simulink subsystem "BatteryHV_Primitive_refsub"  (R2025a)
settings: Solver=VariableStepAuto  StartTime=0.0  StopTime=10.0  RelTol=1e-3
undefined symbols (not defined in the file or in its folder): batteryHV, Minus, Plus
libraries: fl_lib x14, nesl_utility x6
settings Model: Creator=isaacito  LastModifiedBy=isaacito
settings SolverCC: AlgebraicLoopSolver=TrustRegion
settings OptimizationCC: ReuseModelBlockBuffer=off
settings DebuggingCC: UnconnectedInputMsg=warning  UnconnectedOutputMsg=warning  UnconnectedLineMsg=warning
settings ModelReferenceCC: EnableRefExpFcnMdlSchedulingChecks=on
settings RTWCC: GPUComputeCapability=3.5  DLArmComputeVersion=19.05

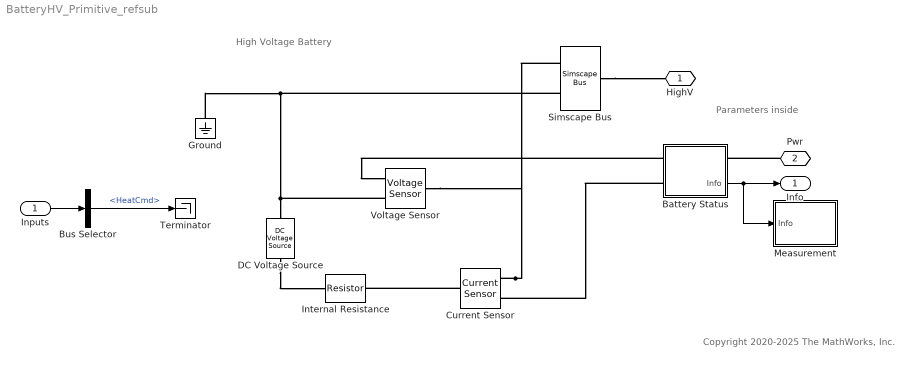
== system BatteryHV_Primitive_refsub ==
  note: Parameters inside
  note: High Voltage Battery
  note: Copyright 2020-2025 The MathWorks, Inc.
  Inputs : Inport
  Battery Status : Subsystem
      settings: PortSchema="{\"entries\":[{\"content\":{\"sides\":[{\"content\":{\"connectorIds\":[\"LConn1\",\"LConn2\"]},\"type\":\"ConnectorPlacement.EquallySpacedRectSide\",\"uuid\":\"fa3fe2c3-d9c0-40ca-976a-fdfa614694fc\"},{\"content\":{\"connectorIds\":[\"RConn1\",\"Out1\"],\"side\":\"RIGHT\"},\"type\":\"ConnectorPlacement.EquallySpacedRectSide\",\"uuid\":\"d6ed96ef-770b-4a18-8b31-ef7e8f253069\"},{\"content\":{\"side\":\"TOP\"},\"type\":\"ConnectorPlacement.EquallySpacedRectSide\",\"uuid\":\"d9a8161e-0196-4518-8226-4ae50c8bd457\"}]},\"type\":\"ConnectorPlacement.EquallySpacedConnector\",\"uuid\":\"0aac0953-a631-4fd0-93f3-a84e629f2b58\"}],\"packageUris\":[\"http://schema.mathworks.com/mf0/Connector/R2020b\"],\"version\":\"1.0\"}"
  Bus Selector : BusSelector  OutputSignals=HeatCmd
  Current Sensor : fl_lib/Electrical/Electrical Sensors/Current Sensor
  DC Voltage Source : fl_lib/Electrical/Electrical Sources/DC Voltage Source  v0=batteryHV.nominalVoltage_V V
      settings: AttributesFormatString=%<v0> [%<v0_unit>]
  Ground : fl_lib/Electrical/Electrical Elements/Electrical Reference
  Internal Resistance : fl_lib/Electrical/Electrical Elements/Resistor  R=batteryHV.internalResistance_Ohm Ohm  i_specify=off  i_priority=High  i=0 A  i_nominal_specify=off  i_nominal_value=1  i_nominal_unit=A  v_specify=off  v_priority=High  v=0 V  v_nominal_specify=off  v_nominal_value=1  v_nominal_unit=V
      settings: AttributesFormatString=%<R> [%<R_unit>]
  Measurement : Subsystem
  Simscape Bus : SimscapeBus  HierarchyStrings=Plus;Minus  ConnectionType=Bus: Bus_HighVoltage
      settings: AttributesFormatString=%<ConnectionType>
  Terminator : Terminator
  Voltage Sensor : fl_lib/Electrical/Electrical Sensors/Voltage Sensor
  HighV : PMIOPort  Side=Right
  Pwr : PMIOPort  Port=2  Side=Right
  Info : Outport
  wires:
  Battery Status/1(Info) -> Measurement/1(Info), Info/1
  Inputs/1 -> Bus Selector/1
  Bus Selector/1 -> Terminator/1  "<HeatCmd>"
  connections:
  Ground/LConn1 -- DC Voltage Source/RConn1 -- Voltage Sensor/RConn2 -- Simscape Bus/LConn2
  Current Sensor/RConn2 -- Simscape Bus/LConn1 -- Voltage Sensor/LConn1
  Battery Status/LConn2 -- Current Sensor/RConn1
  Current Sensor/LConn1 -- Internal Resistance/RConn1
  DC Voltage Source/LConn1 -- Internal Resistance/LConn1
  Battery Status/LConn1 -- Voltage Sensor/RConn1
  Simscape Bus/RConn1 -- HighV/RConn1
  Pwr/RConn1 -- Battery Status/RConn1

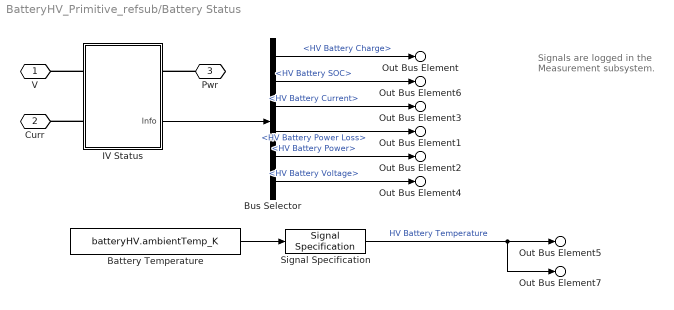
== system BatteryHV_Primitive_refsub/Battery Status ==
  note: Signals are logged in
      | the Measurement subsystem.
  Battery Temperature : Constant  Value=batteryHV.ambientTemp_K
  Bus Selector : BusSelector  OutputSignals=HV Battery Charge,HV Battery SOC,HV Battery Current,HV Battery Power Loss,HV Battery Power,HV Battery Voltage
  IV Status : Subsystem
      settings: PortSchema="{\"entries\":[{\"content\":{\"sides\":[{\"content\":{\"connectorIds\":[\"LConn1\",\"LConn2\"]},\"type\":\"ConnectorPlacement.EquallySpacedRectSide\",\"uuid\":\"fa3fe2c3-d9c0-40ca-976a-fdfa614694fc\"},{\"content\":{\"connectorIds\":[\"RConn1\",\"Out1\"],\"side\":\"RIGHT\"},\"type\":\"ConnectorPlacement.EquallySpacedRectSide\",\"uuid\":\"d6ed96ef-770b-4a18-8b31-ef7e8f253069\"},{\"content\":{\"side\":\"TOP\"},\"type\":\"ConnectorPlacement.EquallySpacedRectSide\",\"uuid\":\"d9a8161e-0196-4518-8226-4ae50c8bd457\"}]},\"type\":\"ConnectorPlacement.EquallySpacedConnector\",\"uuid\":\"0aac0953-a631-4fd0-93f3-a84e629f2b58\"}],\"packageUris\":[\"http://schema.mathworks.com/mf0/Connector/R2020b\"],\"version\":\"1.0\"}"
  Signal Specification : SignalSpecification  Unit=degC
  V : PMIOPort  Side=Left
  Curr : PMIOPort  Port=2  Side=Left
  Pwr : PMIOPort  Port=3  Side=Right
  Out Bus Element5 : Outport  PortName=Info  Element=Temp
  Out Bus Element7 : Outport  PortName=Info  Element=TempAmb
  Out Bus Element : Outport  PortName=Info  Element=Charge
  Out Bus Element3 : Outport  PortName=Info  Element=Current
  Out Bus Element1 : Outport  PortName=Info  Element=PowerLoss
  Out Bus Element2 : Outport  PortName=Info  Element=Power
  Out Bus Element4 : Outport  PortName=Info  Element=Voltage
  Out Bus Element6 : Outport  PortName=Info  Element=SOC
  wires:
  Signal Specification/1 -> Out Bus Element7/1, Out Bus Element5/1  "HV Battery Temperature"
  Battery Temperature/1 -> Signal Specification/1
  Bus Selector/2 -> Out Bus Element6/1  "<HV Battery SOC>"
  Bus Selector/4 -> Out Bus Element1/1  "<HV Battery Power Loss>"
  Bus Selector/1 -> Out Bus Element/1  "<HV Battery Charge>"
  Bus Selector/5 -> Out Bus Element2/1  "<HV Battery Power>"
  Bus Selector/6 -> Out Bus Element4/1  "<HV Battery Voltage>"
  IV Status/1(Info) -> Bus Selector/1
  Bus Selector/3 -> Out Bus Element3/1  "<HV Battery Current>"
  connections:
  Pwr/RConn1 -- IV Status/RConn1
  IV Status/LConn1 -- V/RConn1
  IV Status/LConn2 -- Curr/RConn1

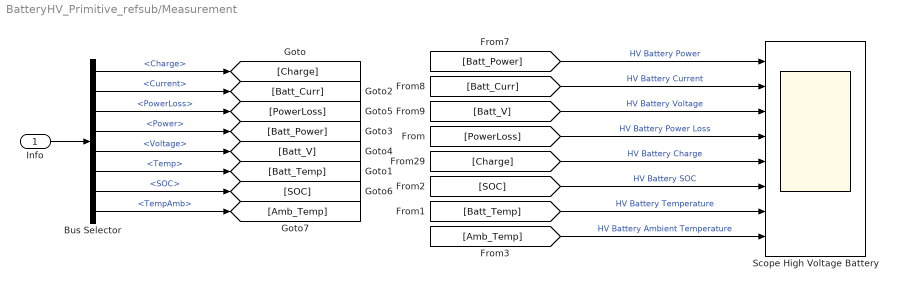
== system BatteryHV_Primitive_refsub/Measurement ==
  Info : Inport
  Bus Selector : BusSelector  OutputSignals=Charge,Current,PowerLoss,Power,Voltage,Temp,SOC,TempAmb
  Scope High Voltage Battery : Scope  NumInputPorts=8
      settings: ActiveDisplayYMinimum=-2.22148  ActiveDisplayYMaximum=4.24683
  wires:
  Bus Selector/1 -> [Charge]  "<Charge>"
  Bus Selector/3 -> [PowerLoss]  "<PowerLoss>"
  Info/1 -> Bus Selector/1
  Bus Selector/5 -> [Batt_V]  "<Voltage>"
  [Batt_Curr] -> Scope High Voltage Battery/2  "HV Battery Current"
  Bus Selector/8 -> [Amb_Temp]  "<TempAmb>"
  [Batt_Power] -> Scope High Voltage Battery/1  "HV Battery Power"
  Bus Selector/6 -> [Batt_Temp]  "<Temp>"
  [Batt_V] -> Scope High Voltage Battery/3  "HV Battery Voltage"
  Bus Selector/4 -> [Batt_Power]  "<Power>"
  Bus Selector/2 -> [Batt_Curr]  "<Current>"
  [PowerLoss] -> Scope High Voltage Battery/4  "HV Battery Power Loss"
  [Charge] -> Scope High Voltage Battery/5  "HV Battery Charge"
  Bus Selector/7 -> [SOC]  "<SOC>"
  [Batt_Temp] -> Scope High Voltage Battery/7  "HV Battery Temperature"
  [Amb_Temp] -> Scope High Voltage Battery/8  "HV Battery Ambient Temperature"
  [SOC] -> Scope High Voltage Battery/6  "HV Battery SOC"

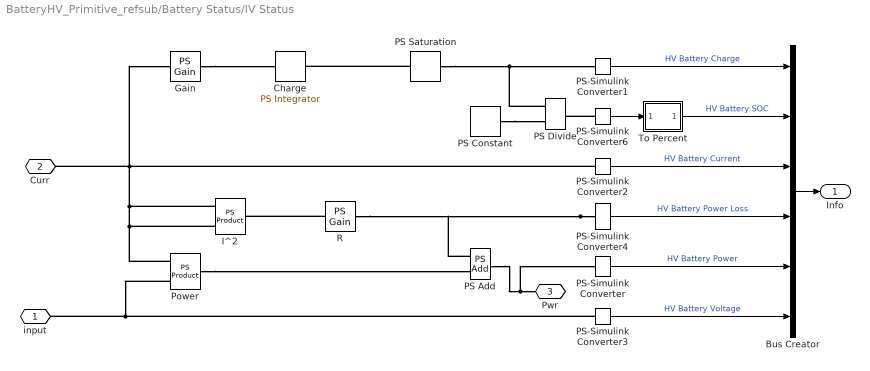
== system BatteryHV_Primitive_refsub/Battery Status/IV Status ==
  Bus Creator : BusCreator  Inputs=6
  Charge : fl_lib/Physical Signals/Linear Operators/PS Integrator  reset_method=foundation.enum.IntegratorResetSpec.None  initial_condition_spec=foundation.enum.IntegratorICSpec.Internal  saturation_spec=foundation.enum.IntegratorSaturationSpec.None  saturation_source_spec=foundation.enum.IntegratorSaturationSourceSpec.Internal  x0=initial.hvBattery_Charge_Ahr A*hr  xu=inf s  xl=-inf s
      settings: AttributesFormatString=%<x0> [%<x0_unit>]
  Gain : fl_lib/Physical Signals/Functions/PS Gain  gain=-1
      settings: AttributesFormatString=%<gain>
  I^2 : fl_lib/Physical Signals/Functions/PS Product
  PS Add : fl_lib/Physical Signals/Functions/PS Add
  PS Constant : fl_lib/Physical Signals/Sources/PS Constant  constant=batteryHV.nominalCharge_Ahr A*hr
      settings: AttributesFormatString=%<constant> [%<constant_unit>]
  PS Divide : fl_lib/Physical Signals/Functions/PS Divide
  PS Saturation : fl_lib/Physical Signals/Nonlinear Operators/PS Saturation  upper_limit=batteryHV.nominalCharge_Ahr A*hr  lower_limit=0 A*hr  ZeroCross=true
      settings: AttributesFormatString=|
      | Upper: %<upper_limit>
      | Lower: %<lower_limit>
  PS-Simulink Converter : nesl_utility/PS-Simulink Converter  PhysicalDomain=network_engine_domain  SubClassName=ps_output  LeftPortType=input  RightPortType=output  PseudoPeriodic=off  Frequencies=[]  VectorFormat=1-D array  Unit=kW  AffineConversion=off
  PS-Simulink Converter1 : nesl_utility/PS-Simulink Converter  PhysicalDomain=network_engine_domain  SubClassName=ps_output  LeftPortType=input  RightPortType=output  PseudoPeriodic=off  Frequencies=[]  VectorFormat=1-D array  Unit=A*hr  AffineConversion=off
  PS-Simulink Converter2 : nesl_utility/PS-Simulink Converter  PhysicalDomain=network_engine_domain  SubClassName=ps_output  LeftPortType=input  RightPortType=output  PseudoPeriodic=off  Frequencies=[]  VectorFormat=1-D array  Unit=A  AffineConversion=off
  PS-Simulink Converter3 : nesl_utility/PS-Simulink Converter  PhysicalDomain=network_engine_domain  SubClassName=ps_output  LeftPortType=input  RightPortType=output  PseudoPeriodic=off  Frequencies=[]  VectorFormat=1-D array  Unit=V  AffineConversion=off
  PS-Simulink Converter4 : nesl_utility/PS-Simulink Converter  PhysicalDomain=network_engine_domain  SubClassName=ps_output  LeftPortType=input  RightPortType=output  PseudoPeriodic=off  Frequencies=[]  VectorFormat=1-D array  Unit=W  AffineConversion=off
  PS-Simulink Converter6 : nesl_utility/PS-Simulink Converter  PhysicalDomain=network_engine_domain  SubClassName=ps_output  LeftPortType=input  RightPortType=output  PseudoPeriodic=off  Frequencies=[]  VectorFormat=1-D array  Unit=1  AffineConversion=off
  Power : fl_lib/Physical Signals/Functions/PS Product
  R : fl_lib/Physical Signals/Functions/PS Gain  gain=batteryHV.internalResistance_Ohm Ohm
      settings: AttributesFormatString=%<gain> [%<gain_unit>]
  To Percent : Subsystem
  input : PMIOPort  Side=Left
  Curr : PMIOPort  Port=2  Side=Left
  Pwr : PMIOPort  Port=3  Side=Right
  Info : Outport
  wires:
  To Percent/1(Out1) -> Bus Creator/2  "HV Battery SOC"
  PS-Simulink Converter4/1 -> Bus Creator/4  "HV Battery Power Loss"
  PS-Simulink Converter3/1 -> Bus Creator/6  "HV Battery Voltage"
  PS-Simulink Converter1/1 -> Bus Creator/1  "HV Battery Charge"
  PS-Simulink Converter6/1 -> To Percent/1(In1)
  PS-Simulink Converter2/1 -> Bus Creator/3  "HV Battery Current"
  PS-Simulink Converter/1 -> Bus Creator/5  "HV Battery Power"
  Bus Creator/1 -> Info/1
  connections:
  Pwr/RConn1 -- PS Add/RConn1 -- PS-Simulink Converter/LConn1
  Power/RConn1 -- PS Add/LConn2
  PS Saturation/LConn1 -- Charge/RConn1
  PS Divide/LConn1 -- PS-Simulink Converter1/LConn1 -- PS Saturation/RConn1
  Power/LConn2 -- I^2/LConn1 -- I^2/LConn2 -- PS-Simulink Converter2/LConn1 -- Gain/LConn1 -- Curr/RConn1
  Power/LConn1 -- PS-Simulink Converter3/LConn1 -- input/RConn1
  PS Constant/RConn1 -- PS Divide/LConn2
  Gain/RConn1 -- Charge/LConn1
  PS-Simulink Converter6/LConn1 -- PS Divide/RConn1
  R/LConn1 -- I^2/RConn1
  PS-Simulink Converter4/LConn1 -- R/RConn1 -- PS Add/LConn1

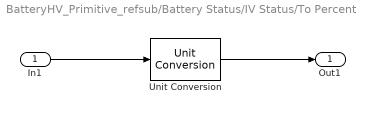
== system BatteryHV_Primitive_refsub/Battery Status/IV Status/To Percent ==
  In1 : Inport
  Unit Conversion : UnitConversion
  Out1 : Outport  Unit=%
      settings: AttributesFormatString=%<Unit>
  wires:
  In1/1 -> Unit Conversion/1
  Unit Conversion/1 -> Out1/1
